simulink model "Simulink_Intro"  (R2026b)
settings: Solver=VariableStepAuto
libraries: simulink x1
settings Model: Creator=nroberts  LastModifiedBy=grant
settings RTWCC: GPUComputeCapability=5.0

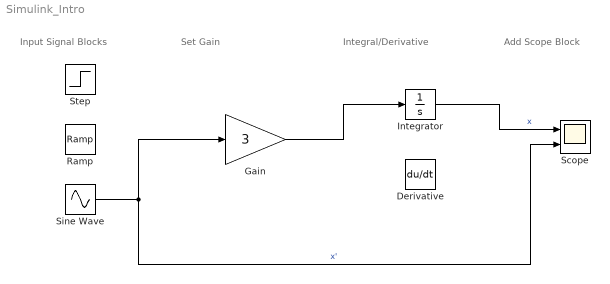
== system Simulink_Intro ==
  note: Add Scope Block
  note: Input Signal Blocks
  note: Set Gain
  note: Integral/Derivative
  Derivative : Derivative
  Gain : Gain  Gain=3
  Integrator : Integrator
  Ramp : simulink/Sources/Ramp  slope=1  start=0  InitialOutput=0
  Scope : Scope  NumInputPorts=2
      settings: ActiveDisplayYMinimum=-1.8705700756571182  ActiveDisplayYMaximum=6.8734845925556733
  Sine Wave : Sin  SampleTime=0
  Step : Step  SampleTime=0
  wires:
  Sine Wave/1 -> Scope/2, Gain/1  "x'"
  Gain/1 -> Integrator/1
  Integrator/1 -> Scope/1  "x"
